simulink model "E1_DifferentialEquation_CT"  (R2024a)
settings: Solver=VariableStepAuto  StartTime=0.0  StopTime=10.0  RelTol=1e-3
settings Model: Creator=Sanagostar  LastModifiedBy=Sanagostar

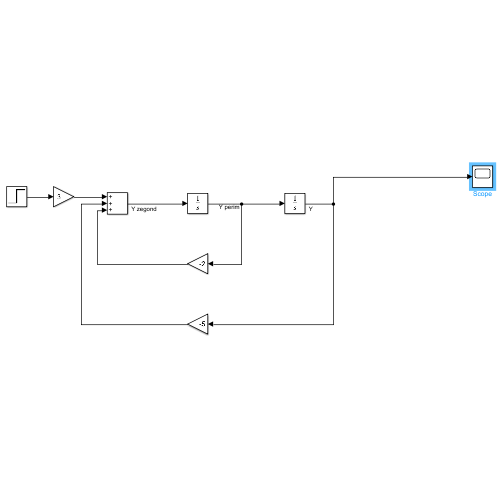
[thumbnail: Simulink's stored preview of the top-level diagram]
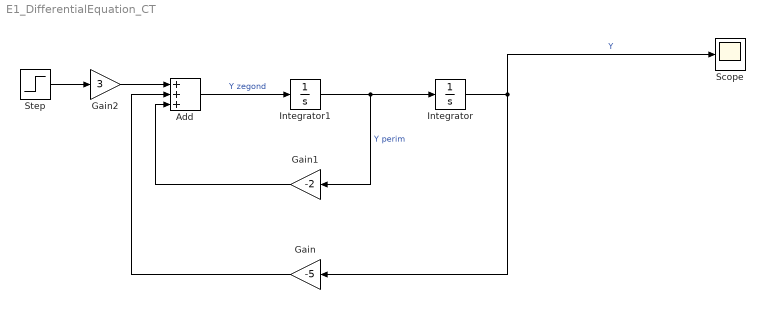
== system E1_DifferentialEquation_CT ==
  Add : Sum  Inputs=+++
  Gain : Gain  Gain=-5
  Gain1 : Gain  Gain=-2
  Gain2 : Gain  Gain=3
  Integrator : Integrator  InitialCondition=1
  Integrator1 : Integrator  InitialCondition=-2
  Scope : Scope
  Step : Step  Time=0  SampleTime=0
  wires:
  Add/1 -> Integrator1/1  "Y zegond"
  Integrator1/1 -> Gain1/1, Integrator/1  "Y perim"
  Gain1/1 -> Add/3
  Gain/1 -> Add/2
  Integrator/1 -> Gain/1, Scope/1  "Y"
  Step/1 -> Gain2/1
  Gain2/1 -> Add/1
